simulink model "generic_IVS"  (R2024a)
settings: Solver=FixedStepDiscrete  StartTime=0.0  StopTime=inf  FixedStep=0.001  RelTol=1e-3  EnableMultiTasking=on
libraries: simulink x1, CarMaker4SL x1
(part 2 of 2)

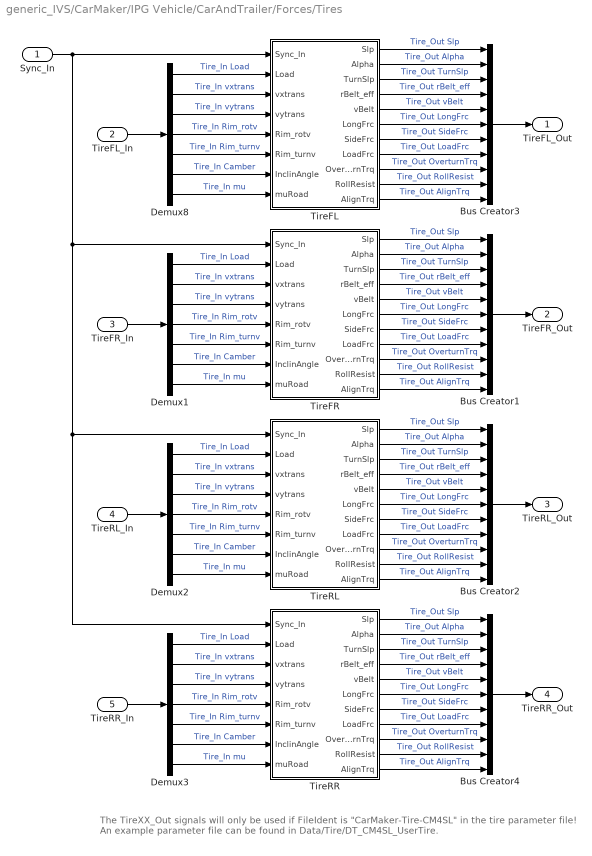
== system generic_IVS/CarMaker/IPG Vehicle/CarAndTrailer/Forces/Tires ==
  note: The TireXX_Out signals will only be used if FileIdent is "CarMaker-Tire-CM4SL" in the tire parameter file!
      | An example parameter file can be found in Data/Tire/DT_CM4SL_UserTire.
  Sync_In : Inport
  TireFL_In : Inport  Port=2
  TireFR_In : Inport  Port=3
  TireRL_In : Inport  Port=4
  TireRR_In : Inport  Port=5
  Bus Creator{1..4} (4 alike) : BusCreator  Inputs=11
  Demux{1..3,8} (4 alike) : Demux  Outputs=7
      settings: DisplayOption=none
  TireFL : Subsystem
  TireFR : Subsystem
  TireRL : Subsystem
  TireRR : Subsystem
  TireFL_Out : Outport  VectorParamsAs1DForOutWhenUnconnected=off
  TireFR_Out : Outport  Port=2  VectorParamsAs1DForOutWhenUnconnected=off
  TireRL_Out : Outport  Port=3  VectorParamsAs1DForOutWhenUnconnected=off
  TireRR_Out : Outport  Port=4  VectorParamsAs1DForOutWhenUnconnected=off
  wires:
  Sync_In/1 -> TireRR/1(Sync_In), TireRL/1(Sync_In), TireFR/1(Sync_In), TireFL/1(Sync_In)
  Bus Creator4/1 -> TireRR_Out/1
  Bus Creator2/1 -> TireRL_Out/1
  Bus Creator1/1 -> TireFR_Out/1
  Demux3/5 -> TireRR/6(Rim_turnv)  "Tire_In Rim_turnv"
  Demux3/4 -> TireRR/5(Rim_rotv)  "Tire_In Rim_rotv"
  Demux3/1 -> TireRR/2(Load)  "Tire_In Load"
  Demux3/7 -> TireRR/8(muRoad)  "Tire_In mu"
  Demux3/6 -> TireRR/7(InclinAngle)  "Tire_In Camber"
  Demux3/2 -> TireRR/3(vxtrans)  "Tire_In vxtrans"
  Demux3/3 -> TireRR/4(vytrans)  "Tire_In vytrans"
  TireRR/11(AlignTrq) -> Bus Creator4/11  "Tire_Out AlignTrq"
  TireRR/10(RollResist) -> Bus Creator4/10  "Tire_Out RollResist"
  TireRR/9(OverturnTrq) -> Bus Creator4/9  "Tire_Out OverturnTrq"
  TireRR/8(LoadFrc) -> Bus Creator4/8  "Tire_Out LoadFrc"
  TireRR/7(SideFrc) -> Bus Creator4/7  "Tire_Out SideFrc"
  TireRR/6(LongFrc) -> Bus Creator4/6  "Tire_Out LongFrc"
  TireRR/5(vBelt) -> Bus Creator4/5  "Tire_Out vBelt"
  TireRR/4(rBelt_eff) -> Bus Creator4/4  "Tire_Out rBelt_eff"
  TireRR/3(TurnSlp) -> Bus Creator4/3  "Tire_Out TurnSlp"
  TireRR/1(Slp) -> Bus Creator4/1  "Tire_Out Slp"
  TireRR/2(Alpha) -> Bus Creator4/2  "Tire_Out Alpha"
  Demux2/5 -> TireRL/6(Rim_turnv)  "Tire_In Rim_turnv"
  Demux2/4 -> TireRL/5(Rim_rotv)  "Tire_In Rim_rotv"
  Demux2/1 -> TireRL/2(Load)  "Tire_In Load"
  Demux2/7 -> TireRL/8(muRoad)  "Tire_In mu"
  Demux2/6 -> TireRL/7(InclinAngle)  "Tire_In Camber"
  Demux2/2 -> TireRL/3(vxtrans)  "Tire_In vxtrans"
  Demux2/3 -> TireRL/4(vytrans)  "Tire_In vytrans"
  TireRL/11(AlignTrq) -> Bus Creator2/11  "Tire_Out AlignTrq"
  TireRL/10(RollResist) -> Bus Creator2/10  "Tire_Out RollResist"
  TireRL/9(OverturnTrq) -> Bus Creator2/9  "Tire_Out OverturnTrq"
  TireRL/8(LoadFrc) -> Bus Creator2/8  "Tire_Out LoadFrc"
  TireRL/7(SideFrc) -> Bus Creator2/7  "Tire_Out SideFrc"
  TireRL/6(LongFrc) -> Bus Creator2/6  "Tire_Out LongFrc"
  TireRL/5(vBelt) -> Bus Creator2/5  "Tire_Out vBelt"
  TireRL/4(rBelt_eff) -> Bus Creator2/4  "Tire_Out rBelt_eff"
  TireRL/3(TurnSlp) -> Bus Creator2/3  "Tire_Out TurnSlp"
  TireRL/1(Slp) -> Bus Creator2/1  "Tire_Out Slp"
  TireRL/2(Alpha) -> Bus Creator2/2  "Tire_Out Alpha"
  Demux1/5 -> TireFR/6(Rim_turnv)  "Tire_In Rim_turnv"
  Demux1/4 -> TireFR/5(Rim_rotv)  "Tire_In Rim_rotv"
  Demux1/1 -> TireFR/2(Load)  "Tire_In Load"
  Demux1/7 -> TireFR/8(muRoad)  "Tire_In mu"
  Demux1/6 -> TireFR/7(InclinAngle)  "Tire_In Camber"
  Demux1/2 -> TireFR/3(vxtrans)  "Tire_In vxtrans"
  Demux1/3 -> TireFR/4(vytrans)  "Tire_In vytrans"
  TireFR/11(AlignTrq) -> Bus Creator1/11  "Tire_Out AlignTrq"
  TireFR/10(RollResist) -> Bus Creator1/10  "Tire_Out RollResist"
  TireFR/9(OverturnTrq) -> Bus Creator1/9  "Tire_Out OverturnTrq"
  TireFR/8(LoadFrc) -> Bus Creator1/8  "Tire_Out LoadFrc"
  TireFR/7(SideFrc) -> Bus Creator1/7  "Tire_Out SideFrc"
  TireFR/6(LongFrc) -> Bus Creator1/6  "Tire_Out LongFrc"
  TireFR/5(vBelt) -> Bus Creator1/5  "Tire_Out vBelt"
  TireFR/4(rBelt_eff) -> Bus Creator1/4  "Tire_Out rBelt_eff"
  TireFR/3(TurnSlp) -> Bus Creator1/3  "Tire_Out TurnSlp"
  TireFR/1(Slp) -> Bus Creator1/1  "Tire_Out Slp"
  TireFR/2(Alpha) -> Bus Creator1/2  "Tire_Out Alpha"
  Demux8/5 -> TireFL/6(Rim_turnv)  "Tire_In Rim_turnv"
  Demux8/4 -> TireFL/5(Rim_rotv)  "Tire_In Rim_rotv"
  TireFL_In/1 -> Demux8/1
  Demux8/1 -> TireFL/2(Load)  "Tire_In Load"
  Demux8/7 -> TireFL/8(muRoad)  "Tire_In mu"
  Demux8/6 -> TireFL/7(InclinAngle)  "Tire_In Camber"
  Demux8/2 -> TireFL/3(vxtrans)  "Tire_In vxtrans"
  Demux8/3 -> TireFL/4(vytrans)  "Tire_In vytrans"
  TireFL/11(AlignTrq) -> Bus Creator3/11  "Tire_Out AlignTrq"
  TireFL/10(RollResist) -> Bus Creator3/10  "Tire_Out RollResist"
  TireFL/9(OverturnTrq) -> Bus Creator3/9  "Tire_Out OverturnTrq"
  TireFL/8(LoadFrc) -> Bus Creator3/8  "Tire_Out LoadFrc"
  TireFL/7(SideFrc) -> Bus Creator3/7  "Tire_Out SideFrc"
  TireFL/6(LongFrc) -> Bus Creator3/6  "Tire_Out LongFrc"
  TireFL/5(vBelt) -> Bus Creator3/5  "Tire_Out vBelt"
  TireFL/4(rBelt_eff) -> Bus Creator3/4  "Tire_Out rBelt_eff"
  TireFL/3(TurnSlp) -> Bus Creator3/3  "Tire_Out TurnSlp"
  TireFL/1(Slp) -> Bus Creator3/1  "Tire_Out Slp"
  TireFL/2(Alpha) -> Bus Creator3/2  "Tire_Out Alpha"
  Bus Creator3/1 -> TireFL_Out/1
  TireFR_In/1 -> Demux1/1
  TireRL_In/1 -> Demux2/1
  TireRR_In/1 -> Demux3/1

== system generic_IVS/CarMaker/IPG Vehicle/CarAndTrailer/Forces/Vehicle Forces ==
  Sync_In : Inport
  Bus Creator1 : BusCreator  Inputs=12
  Bus Creator8 : BusCreator  Inputs=16
  BusCreator1 : BusCreator  Inputs=4
  BusCreator2 : BusCreator  Inputs=9
  Demux : Demux  Outputs=16
      settings: DisplayOption=none
  Demux1 : Demux  Outputs=12
      settings: DisplayOption=none
  Demux2 : Demux  Outputs=13
      settings: DisplayOption=none
  Forces : S-Function  FunctionName=CM_Sfun  Parameters='Forces'  SFunctionDeploymentMode=off  EnableBusSupport=off
  Terminator : Terminator
  Sync_Out : Outport  VectorParamsAs1DForOutWhenUnconnected=off
  Car.Virtual : Outport  Port=2  VectorParamsAs1DForOutWhenUnconnected=off
  Car.Aero : Outport  Port=3  VectorParamsAs1DForOutWhenUnconnected=off
  Car.Load : Outport  Port=4  VectorParamsAs1DForOutWhenUnconnected=off
  wires:
  BusCreator1/1 -> Terminator/1  "Aero IF (in)"
  Demux2/13 -> BusCreator2/9  "car Aero Trq_1 z"
  Demux2/12 -> BusCreator2/8  "car Aero Trq_1 y"
  Demux2/11 -> BusCreator2/7  "car Aero Trq_1 x"
  Demux2/10 -> BusCreator2/6  "car Aero Frc_1 z"
  Demux2/9 -> BusCreator2/5  "car Aero Frc_1 y"
  Demux2/8 -> BusCreator2/4  "car Aero Frc_1 x"
  Demux2/7 -> BusCreator2/3  "car Aero PoA_1 z"
  Demux2/6 -> BusCreator2/2  "car Aero PoA_1 y"
  Demux2/5 -> BusCreator2/1  "car Aero PoA_1 x"
  Demux2/4 -> BusCreator1/4  "car Aero tau_1"
  Demux2/3 -> BusCreator1/3  "car Aero ApproachVel_1 z"
  Demux2/2 -> BusCreator1/2  "car Aero ApproachVel_1 y"
  Demux2/1 -> BusCreator1/1  "car Aero ApproachVel_1 x"
  Demux/16 -> Bus Creator8/16  "Car Load_3 tz"
  Demux/15 -> Bus Creator8/15  "Car Load_3 ty"
  Demux/14 -> Bus Creator8/14  "Car Load_3 tx"
  Demux/13 -> Bus Creator8/13  "Car Load_3 mass"
  Demux1/12 -> Bus Creator1/12  "Car Virtual Trq_0 z"
  Demux1/11 -> Bus Creator1/11  "Car Virtual Trq_0 y"
  Demux1/10 -> Bus Creator1/10  "Car Virtual Trq_0 x"
  Demux1/9 -> Bus Creator1/9  "Car Virtual Trq_1 z"
  Demux1/8 -> Bus Creator1/8  "Car Virtual Trq_1 y"
  Demux1/7 -> Bus Creator1/7  "Car Virtual Trq_1 x"
  Demux1/6 -> Bus Creator1/6  "Car Virtual Frc_0 z"
  Demux1/5 -> Bus Creator1/5  "Car Virtual Frc_0 y"
  Demux1/4 -> Bus Creator1/4  "Car Virtual Frc_0 x"
  Sync_In/1 -> Forces/1
  Forces/1 -> Sync_Out/1
  BusCreator2/1 -> Car.Aero/1
  Demux1/1 -> Bus Creator1/1  "Car Virtual Frc_1 x"
  Demux1/2 -> Bus Creator1/2  "Car Virtual Frc_1 y"
  Demux1/3 -> Bus Creator1/3  "Car Virtual Frc_1 z"
  Forces/3 -> Demux2/1
  Forces/2 -> Demux1/1
  Bus Creator1/1 -> Car.Virtual/1
  Bus Creator8/1 -> Car.Load/1
  Demux/1 -> Bus Creator8/1  "Car Load_0 mass"
  Demux/2 -> Bus Creator8/2  "Car Load_0 tx"
  Demux/3 -> Bus Creator8/3  "Car Load_0 ty"
  Demux/4 -> Bus Creator8/4  "Car Load_0 tz"
  Demux/5 -> Bus Creator8/5  "Car Load_1 mass"
  Demux/6 -> Bus Creator8/6  "Car Load_1 tx"
  Demux/7 -> Bus Creator8/7  "Car Load_1 ty"
  Demux/8 -> Bus Creator8/8  "Car Load_1 tz"
  Demux/9 -> Bus Creator8/9  "Car Load_2 mass"
  Demux/10 -> Bus Creator8/10  "Car Load_2 tx"
  Demux/11 -> Bus Creator8/11  "Car Load_2 ty"
  Demux/12 -> Bus Creator8/12  "Car Load_2 tz"
  Forces/4 -> Demux/1

== system generic_IVS/CarMaker/IPG Vehicle/CarAndTrailer/Trailer/CreateBus Car.Hitch.FrcTrq ==
  In1 : Inport
  Bus Creator7 : BusCreator  Inputs=6
  Demux7 : Demux  Outputs=6
      settings: DisplayOption=none
  Out1 : Outport  VectorParamsAs1DForOutWhenUnconnected=off
  wires:
  In1/1 -> Demux7/1
  Bus Creator7/1 -> Out1/1
  Demux7/6 -> Bus Creator7/6  "Car Hitch Trq2Car z"
  Demux7/5 -> Bus Creator7/5  "Car Hitch Trq2Car y"
  Demux7/4 -> Bus Creator7/4  "Car Hitch Trq2Car x"
  Demux7/3 -> Bus Creator7/3  "Car Hitch Frc2Car z"
  Demux7/2 -> Bus Creator7/2  "Car Hitch Frc2Car y"
  Demux7/1 -> Bus Creator7/1  "Car Hitch Frc2Car x"

== system generic_IVS/CarMaker/IPG Vehicle/CarAndTrailer/Trailer/CreateBus Vhcl.Motion ==
  In1 : Inport
  BusCreator : BusCreator  Inputs=15
  Demux : Demux  Outputs=15
      settings: DisplayOption=none
  Out1 : Outport  VectorParamsAs1DForOutWhenUnconnected=off
  wires:
  Demux/15 -> BusCreator/15  "Vhcl YawAcc"
  Demux/14 -> BusCreator/14  "Vhcl YawVel"
  Demux/13 -> BusCreator/13  "Vhcl Yaw"
  Demux/12 -> BusCreator/12  "Vhcl PitchAcc"
  Demux/11 -> BusCreator/11  "Vhcl PitchVel"
  Demux/10 -> BusCreator/10  "Vhcl Pitch"
  Demux/9 -> BusCreator/9  "Vhcl RollAcc"
  Demux/8 -> BusCreator/8  "Vhcl RollVel"
  Demux/7 -> BusCreator/7  "Vhcl Roll"
  Demux/6 -> BusCreator/6  "Vhcl Hitch_Pos z"
  Demux/5 -> BusCreator/5  "Vhcl Hitch_Pos y"
  Demux/4 -> BusCreator/4  "Vhcl Hitch_Pos x"
  Demux/3 -> BusCreator/3  "Vhcl sRoad"
  Demux/2 -> BusCreator/2  "Vhcl Distance"
  Demux/1 -> BusCreator/1  "Vhcl v"
  In1/1 -> Demux/1
  BusCreator/1 -> Out1/1

== system generic_IVS/CarMaker/IPG Vehicle/CarAndTrailer/Trailer/CreateBus Vhcl.PoI ==
  In1 : Inport
  Bus Creator3 : BusCreator  Inputs=18
  Demux3 : Demux  Outputs=18
      settings: DisplayOption=none
  Out1 : Outport  VectorParamsAs1DForOutWhenUnconnected=off
  wires:
  Demux3/18 -> Bus Creator3/18  "Vhcl PoI_GCS Elev"
  Demux3/17 -> Bus Creator3/17  "Vhcl PoI_GCS Lat"
  Demux3/16 -> Bus Creator3/16  "Vhcl PoI_GCS Long"
  Demux3/15 -> Bus Creator3/15  "Vhcl PoI_Acc_1 z"
  Demux3/14 -> Bus Creator3/14  "Vhcl PoI_Acc_1 y"
  Demux3/13 -> Bus Creator3/13  "Vhcl PoI_Acc_1 x"
  Demux3/12 -> Bus Creator3/12  "Vhcl PoI_Vel_1 z"
  Demux3/11 -> Bus Creator3/11  "Vhcl PoI_Vel_1 y"
  Demux3/10 -> Bus Creator3/10  "Vhcl PoI_Vel_1 x"
  Demux3/9 -> Bus Creator3/9  "Vhcl PoI_Acc z"
  Demux3/8 -> Bus Creator3/8  "Vhcl PoI_Acc y"
  Demux3/7 -> Bus Creator3/7  "Vhcl PoI_Acc x"
  Demux3/6 -> Bus Creator3/6  "Vhcl PoI_Vel z"
  Demux3/5 -> Bus Creator3/5  "Vhcl PoI_Vel y"
  Demux3/4 -> Bus Creator3/4  "Vhcl PoI_Vel x"
  Demux3/3 -> Bus Creator3/3  "Vhcl PoI_Pos z"
  Demux3/2 -> Bus Creator3/2  "Vhcl PoI_Pos y"
  In1/1 -> Demux3/1
  Bus Creator3/1 -> Out1/1
  Demux3/1 -> Bus Creator3/1  "Vhcl PoI_Pos x"

== system generic_IVS/CarMaker/IPG Vehicle/CarAndTrailer/Trailer/CreateBus Vhcl.Steering ==
  In1 : Inport
  Bus Creator3 : BusCreator  Inputs=4
  Demux : Demux
      settings: DisplayOption=none
  Out1 : Outport  VectorParamsAs1DForOutWhenUnconnected=off
  wires:
  Bus Creator3/1 -> Out1/1
  Demux/1 -> Bus Creator3/1  "Vhcl Steering Ang"
  Demux/3 -> Bus Creator3/3  "Vhcl Steering AngAcc"
  Demux/2 -> Bus Creator3/2  "Vhcl Steering AngVel"
  Demux/4 -> Bus Creator3/4  "Vhcl Steering Trq"
  In1/1 -> Demux/1

== system generic_IVS/CarMaker/IPG Vehicle/CarAndTrailer/Trailer/CreateBus Vhcl.Wheel.FL ==
  In1 : Inport
  Bus Creator3 : BusCreator  Inputs=14
  Demux3 : Demux  Outputs=14
      settings: DisplayOption=none
  Out1 : Outport  VectorParamsAs1DForOutWhenUnconnected=off
  wires:
  Demux3/14 -> Bus Creator3/14  "Vhcl Wheel FL Trq_WhlBearing"
  Demux3/13 -> Bus Creator3/13  "Vhcl Wheel FL Trq_T2W"
  Demux3/12 -> Bus Creator3/12  "Vhcl Wheel FL SideSlip"
  Demux3/11 -> Bus Creator3/11  "Vhcl Wheel FL LongSlip"
  Demux3/10 -> Bus Creator3/10  "Vhcl Wheel FL vBelt"
  Demux3/9 -> Bus Creator3/9  "Vhcl Wheel FL Fz"
  Demux3/8 -> Bus Creator3/8  "Vhcl Wheel FL Fy"
  Demux3/7 -> Bus Creator3/7  "Vhcl Wheel FL Fx"
  Demux3/6 -> Bus Creator3/6  "Vhcl Wheel FL r_zxy z"
  Demux3/5 -> Bus Creator3/5  "Vhcl Wheel FL r_zxy y"
  Demux3/4 -> Bus Creator3/4  "Vhcl Wheel FL r_zxy x"
  Demux3/3 -> Bus Creator3/3  "Vhcl Wheel FL t z"
  Demux3/2 -> Bus Creator3/2  "Vhcl Wheel FL t y"
  In1/1 -> Demux3/1
  Bus Creator3/1 -> Out1/1
  Demux3/1 -> Bus Creator3/1  "Vhcl Wheel FL t x"

== system generic_IVS/CarMaker/IPG Vehicle/CarAndTrailer/Trailer/CreateBus Vhcl.Wheel.FR ==
  In1 : Inport
  Bus Creator3 : BusCreator  Inputs=14
  Demux3 : Demux  Outputs=14
      settings: DisplayOption=none
  Out1 : Outport  VectorParamsAs1DForOutWhenUnconnected=off
  wires:
  Demux3/14 -> Bus Creator3/14  "Vhcl Wheel FR Trq_WhlBearing"
  Demux3/13 -> Bus Creator3/13  "Vhcl Wheel FR Trq_T2W"
  Demux3/12 -> Bus Creator3/12  "Vhcl Wheel FR SideSlip"
  Demux3/11 -> Bus Creator3/11  "Vhcl Wheel FR LongSlip"
  Demux3/10 -> Bus Creator3/10  "Vhcl Wheel FR vBelt"
  Demux3/9 -> Bus Creator3/9  "Vhcl Wheel FR Fz"
  Demux3/8 -> Bus Creator3/8  "Vhcl Wheel FR Fy"
  Demux3/7 -> Bus Creator3/7  "Vhcl Wheel FR Fx"
  Demux3/6 -> Bus Creator3/6  "Vhcl Wheel FR r_zxy z"
  Demux3/5 -> Bus Creator3/5  "Vhcl Wheel FR r_zxy y"
  Demux3/4 -> Bus Creator3/4  "Vhcl Wheel FR r_zxy x"
  Demux3/3 -> Bus Creator3/3  "Vhcl Wheel FR t z"
  Demux3/2 -> Bus Creator3/2  "Vhcl Wheel FR t y"
  In1/1 -> Demux3/1
  Bus Creator3/1 -> Out1/1
  Demux3/1 -> Bus Creator3/1  "Vhcl Wheel FR t x"

== system generic_IVS/CarMaker/IPG Vehicle/CarAndTrailer/Trailer/CreateBus Vhcl.Wheel.RL ==
  In1 : Inport
  Bus Creator3 : BusCreator  Inputs=14
  Demux3 : Demux  Outputs=14
      settings: DisplayOption=none
  Out1 : Outport  VectorParamsAs1DForOutWhenUnconnected=off
  wires:
  Demux3/14 -> Bus Creator3/14  "Vhcl Wheel RL Trq_WhlBearing"
  Demux3/13 -> Bus Creator3/13  "Vhcl Wheel RL Trq_T2W"
  Demux3/12 -> Bus Creator3/12  "Vhcl Wheel RL SideSlip"
  Demux3/11 -> Bus Creator3/11  "Vhcl Wheel RL LongSlip"
  Demux3/10 -> Bus Creator3/10  "Vhcl Wheel RL vBelt"
  Demux3/9 -> Bus Creator3/9  "Vhcl Wheel RL Fz"
  Demux3/8 -> Bus Creator3/8  "Vhcl Wheel RL Fy"
  Demux3/7 -> Bus Creator3/7  "Vhcl Wheel RL Fx"
  Demux3/6 -> Bus Creator3/6  "Vhcl Wheel RL r_zxy z"
  Demux3/5 -> Bus Creator3/5  "Vhcl Wheel RL r_zxy y"
  Demux3/4 -> Bus Creator3/4  "Vhcl Wheel RL r_zxy x"
  Demux3/3 -> Bus Creator3/3  "Vhcl Wheel RL t z"
  Demux3/2 -> Bus Creator3/2  "Vhcl Wheel RL t y"
  In1/1 -> Demux3/1
  Bus Creator3/1 -> Out1/1
  Demux3/1 -> Bus Creator3/1  "Vhcl Wheel RL t x"

== system generic_IVS/CarMaker/IPG Vehicle/CarAndTrailer/Trailer/CreateBus Vhcl.Wheel.RR ==
  In1 : Inport
  Bus Creator3 : BusCreator  Inputs=14
  Demux3 : Demux  Outputs=14
      settings: DisplayOption=none
  Out1 : Outport  VectorParamsAs1DForOutWhenUnconnected=off
  wires:
  Demux3/14 -> Bus Creator3/14  "Vhcl Wheel RR Trq_WhlBearing"
  Demux3/13 -> Bus Creator3/13  "Vhcl Wheel RR Trq_T2W"
  Demux3/12 -> Bus Creator3/12  "Vhcl Wheel RR SideSlip"
  Demux3/11 -> Bus Creator3/11  "Vhcl Wheel RR LongSlip"
  Demux3/10 -> Bus Creator3/10  "Vhcl Wheel RR vBelt"
  Demux3/9 -> Bus Creator3/9  "Vhcl Wheel RR Fz"
  Demux3/8 -> Bus Creator3/8  "Vhcl Wheel RR Fy"
  Demux3/7 -> Bus Creator3/7  "Vhcl Wheel RR Fx"
  Demux3/6 -> Bus Creator3/6  "Vhcl Wheel RR r_zxy z"
  Demux3/5 -> Bus Creator3/5  "Vhcl Wheel RR r_zxy y"
  Demux3/4 -> Bus Creator3/4  "Vhcl Wheel RR r_zxy x"
  Demux3/3 -> Bus Creator3/3  "Vhcl Wheel RR t z"
  Demux3/2 -> Bus Creator3/2  "Vhcl Wheel RR t y"
  In1/1 -> Demux3/1
  Bus Creator3/1 -> Out1/1
  Demux3/1 -> Bus Creator3/1  "Vhcl Wheel RR t x"

== system generic_IVS/CarMaker/IPG Vehicle/CarAndTrailer/Forces/Suspension Forces/Suspension External Forces Update ==
  Bus Creator21 : BusCreator  Inputs=6
  Bus Creator22 : BusCreator  Inputs=4
  Bus Creator23 : BusCreator  Inputs=4
  From : From  TagVisibility=global
  Ground{32..39} (8 alike) : Ground
  Out1 : Outport
  wires:
  [D] -> Bus Creator21/4
  Ground36/1 -> Bus Creator22/1
  From/1 -> Bus Creator21/1
  [B] -> Bus Creator21/2
  Ground34/1 -> Bus Creator23/3
  Ground32/1 -> Bus Creator23/1
  [C] -> Bus Creator21/3
  Bus Creator23/1 -> Bus Creator21/5
  Ground33/1 -> Bus Creator23/2
  Bus Creator22/1 -> Bus Creator21/6
  Bus Creator21/1 -> Out1/1
  Ground35/1 -> Bus Creator23/4
  Ground39/1 -> Bus Creator22/4
  Ground38/1 -> Bus Creator22/3
  Ground37/1 -> Bus Creator22/2

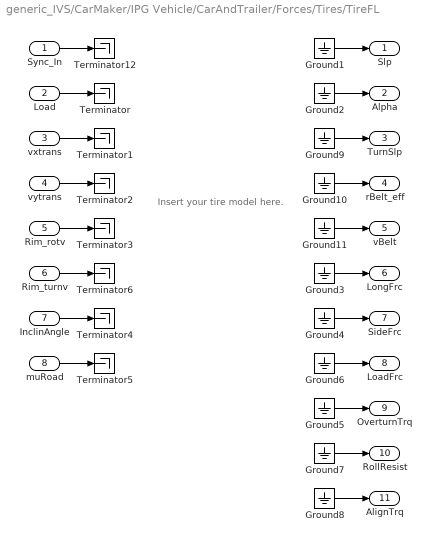
== system generic_IVS/CarMaker/IPG Vehicle/CarAndTrailer/Forces/Tires/TireFL ==
  note: Insert your tire model here.
  Sync_In : Inport
  Load : Inport  Port=2
  vxtrans : Inport  Port=3
  vytrans : Inport  Port=4
  Rim_rotv : Inport  Port=5
  Rim_turnv : Inport  Port=6
  InclinAngle : Inport  Port=7
  muRoad : Inport  Port=8
  Ground{1..11} (11 alike) : Ground
  Terminator{,1..6,12} (8 alike) : Terminator
  Slp : Outport  VectorParamsAs1DForOutWhenUnconnected=off
  Alpha : Outport  Port=2  VectorParamsAs1DForOutWhenUnconnected=off
  TurnSlp : Outport  Port=3  VectorParamsAs1DForOutWhenUnconnected=off
  rBelt_eff : Outport  Port=4  VectorParamsAs1DForOutWhenUnconnected=off
  vBelt : Outport  Port=5  VectorParamsAs1DForOutWhenUnconnected=off
  LongFrc : Outport  Port=6  VectorParamsAs1DForOutWhenUnconnected=off
  SideFrc : Outport  Port=7  VectorParamsAs1DForOutWhenUnconnected=off
  LoadFrc : Outport  Port=8  VectorParamsAs1DForOutWhenUnconnected=off
  OverturnTrq : Outport  Port=9  VectorParamsAs1DForOutWhenUnconnected=off
  RollResist : Outport  Port=10  VectorParamsAs1DForOutWhenUnconnected=off
  AlignTrq : Outport  Port=11  VectorParamsAs1DForOutWhenUnconnected=off
  wires:
  Ground11/1 -> vBelt/1
  Ground10/1 -> rBelt_eff/1
  Ground9/1 -> TurnSlp/1
  Rim_turnv/1 -> Terminator6/1
  Sync_In/1 -> Terminator12/1
  Ground2/1 -> Alpha/1
  Ground3/1 -> LongFrc/1
  Ground4/1 -> SideFrc/1
  Ground5/1 -> OverturnTrq/1
  vxtrans/1 -> Terminator1/1
  vytrans/1 -> Terminator2/1
  Rim_rotv/1 -> Terminator3/1
  InclinAngle/1 -> Terminator4/1
  muRoad/1 -> Terminator5/1
  Load/1 -> Terminator/1
  Ground1/1 -> Slp/1
  Ground6/1 -> LoadFrc/1
  Ground7/1 -> RollResist/1
  Ground8/1 -> AlignTrq/1

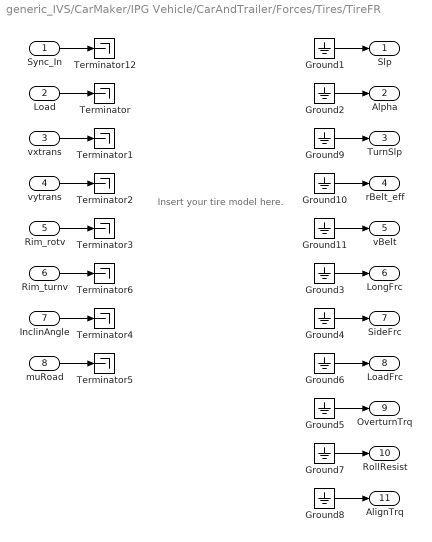
== system generic_IVS/CarMaker/IPG Vehicle/CarAndTrailer/Forces/Tires/TireFR ==
  note: Insert your tire model here.
  Sync_In : Inport
  Load : Inport  Port=2
  vxtrans : Inport  Port=3
  vytrans : Inport  Port=4
  Rim_rotv : Inport  Port=5
  Rim_turnv : Inport  Port=6
  InclinAngle : Inport  Port=7
  muRoad : Inport  Port=8
  Ground{1..11} (11 alike) : Ground
  Terminator{,1..6,12} (8 alike) : Terminator
  Slp : Outport  VectorParamsAs1DForOutWhenUnconnected=off
  Alpha : Outport  Port=2  VectorParamsAs1DForOutWhenUnconnected=off
  TurnSlp : Outport  Port=3  VectorParamsAs1DForOutWhenUnconnected=off
  rBelt_eff : Outport  Port=4  VectorParamsAs1DForOutWhenUnconnected=off
  vBelt : Outport  Port=5  VectorParamsAs1DForOutWhenUnconnected=off
  LongFrc : Outport  Port=6  VectorParamsAs1DForOutWhenUnconnected=off
  SideFrc : Outport  Port=7  VectorParamsAs1DForOutWhenUnconnected=off
  LoadFrc : Outport  Port=8  VectorParamsAs1DForOutWhenUnconnected=off
  OverturnTrq : Outport  Port=9  VectorParamsAs1DForOutWhenUnconnected=off
  RollResist : Outport  Port=10  VectorParamsAs1DForOutWhenUnconnected=off
  AlignTrq : Outport  Port=11  VectorParamsAs1DForOutWhenUnconnected=off
  wires:
  Ground11/1 -> vBelt/1
  Ground10/1 -> rBelt_eff/1
  Ground9/1 -> TurnSlp/1
  Rim_turnv/1 -> Terminator6/1
  Sync_In/1 -> Terminator12/1
  Ground2/1 -> Alpha/1
  Ground3/1 -> LongFrc/1
  Ground4/1 -> SideFrc/1
  Ground5/1 -> OverturnTrq/1
  vxtrans/1 -> Terminator1/1
  vytrans/1 -> Terminator2/1
  Rim_rotv/1 -> Terminator3/1
  InclinAngle/1 -> Terminator4/1
  muRoad/1 -> Terminator5/1
  Load/1 -> Terminator/1
  Ground1/1 -> Slp/1
  Ground6/1 -> LoadFrc/1
  Ground7/1 -> RollResist/1
  Ground8/1 -> AlignTrq/1

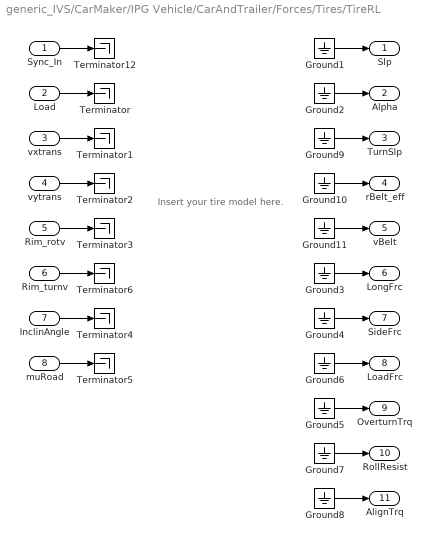
== system generic_IVS/CarMaker/IPG Vehicle/CarAndTrailer/Forces/Tires/TireRL ==
  note: Insert your tire model here.
  Sync_In : Inport
  Load : Inport  Port=2
  vxtrans : Inport  Port=3
  vytrans : Inport  Port=4
  Rim_rotv : Inport  Port=5
  Rim_turnv : Inport  Port=6
  InclinAngle : Inport  Port=7
  muRoad : Inport  Port=8
  Ground{1..11} (11 alike) : Ground
  Terminator{,1..6,12} (8 alike) : Terminator
  Slp : Outport  VectorParamsAs1DForOutWhenUnconnected=off
  Alpha : Outport  Port=2  VectorParamsAs1DForOutWhenUnconnected=off
  TurnSlp : Outport  Port=3  VectorParamsAs1DForOutWhenUnconnected=off
  rBelt_eff : Outport  Port=4  VectorParamsAs1DForOutWhenUnconnected=off
  vBelt : Outport  Port=5  VectorParamsAs1DForOutWhenUnconnected=off
  LongFrc : Outport  Port=6  VectorParamsAs1DForOutWhenUnconnected=off
  SideFrc : Outport  Port=7  VectorParamsAs1DForOutWhenUnconnected=off
  LoadFrc : Outport  Port=8  VectorParamsAs1DForOutWhenUnconnected=off
  OverturnTrq : Outport  Port=9  VectorParamsAs1DForOutWhenUnconnected=off
  RollResist : Outport  Port=10  VectorParamsAs1DForOutWhenUnconnected=off
  AlignTrq : Outport  Port=11  VectorParamsAs1DForOutWhenUnconnected=off
  wires:
  Ground11/1 -> vBelt/1
  Ground10/1 -> rBelt_eff/1
  Ground9/1 -> TurnSlp/1
  Rim_turnv/1 -> Terminator6/1
  Sync_In/1 -> Terminator12/1
  Ground2/1 -> Alpha/1
  Ground3/1 -> LongFrc/1
  Ground4/1 -> SideFrc/1
  Ground5/1 -> OverturnTrq/1
  vxtrans/1 -> Terminator1/1
  vytrans/1 -> Terminator2/1
  Rim_rotv/1 -> Terminator3/1
  InclinAngle/1 -> Terminator4/1
  muRoad/1 -> Terminator5/1
  Load/1 -> Terminator/1
  Ground1/1 -> Slp/1
  Ground6/1 -> LoadFrc/1
  Ground7/1 -> RollResist/1
  Ground8/1 -> AlignTrq/1

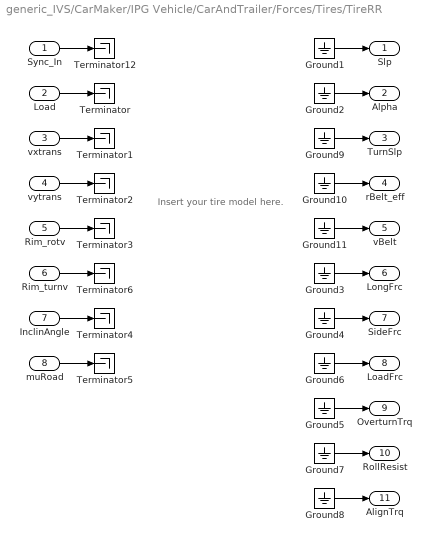
== system generic_IVS/CarMaker/IPG Vehicle/CarAndTrailer/Forces/Tires/TireRR ==
  note: Insert your tire model here.
  Sync_In : Inport
  Load : Inport  Port=2
  vxtrans : Inport  Port=3
  vytrans : Inport  Port=4
  Rim_rotv : Inport  Port=5
  Rim_turnv : Inport  Port=6
  InclinAngle : Inport  Port=7
  muRoad : Inport  Port=8
  Ground{1..11} (11 alike) : Ground
  Terminator{,1..6,12} (8 alike) : Terminator
  Slp : Outport  VectorParamsAs1DForOutWhenUnconnected=off
  Alpha : Outport  Port=2  VectorParamsAs1DForOutWhenUnconnected=off
  TurnSlp : Outport  Port=3  VectorParamsAs1DForOutWhenUnconnected=off
  rBelt_eff : Outport  Port=4  VectorParamsAs1DForOutWhenUnconnected=off
  vBelt : Outport  Port=5  VectorParamsAs1DForOutWhenUnconnected=off
  LongFrc : Outport  Port=6  VectorParamsAs1DForOutWhenUnconnected=off
  SideFrc : Outport  Port=7  VectorParamsAs1DForOutWhenUnconnected=off
  LoadFrc : Outport  Port=8  VectorParamsAs1DForOutWhenUnconnected=off
  OverturnTrq : Outport  Port=9  VectorParamsAs1DForOutWhenUnconnected=off
  RollResist : Outport  Port=10  VectorParamsAs1DForOutWhenUnconnected=off
  AlignTrq : Outport  Port=11  VectorParamsAs1DForOutWhenUnconnected=off
  wires:
  Ground11/1 -> vBelt/1
  Ground10/1 -> rBelt_eff/1
  Ground9/1 -> TurnSlp/1
  Rim_turnv/1 -> Terminator6/1
  Sync_In/1 -> Terminator12/1
  Ground2/1 -> Alpha/1
  Ground3/1 -> LongFrc/1
  Ground4/1 -> SideFrc/1
  Ground5/1 -> OverturnTrq/1
  vxtrans/1 -> Terminator1/1
  vytrans/1 -> Terminator2/1
  Rim_rotv/1 -> Terminator3/1
  InclinAngle/1 -> Terminator4/1
  muRoad/1 -> Terminator5/1
  Load/1 -> Terminator/1
  Ground1/1 -> Slp/1
  Ground6/1 -> LoadFrc/1
  Ground7/1 -> RollResist/1
  Ground8/1 -> AlignTrq/1

== stateflow chart generic_IVS/CarMaker/Subsystem/Day3/Chart ==
  (default) -> (junction 1)
  (junction 1) -> (junction 3) [order 1] : [i<99]
      | {i = i + 1;}
  (junction 1) -> (junction 7) [order 2] : {i=0;}
  (junction 3) -> (junction 5)
  (junction 5) -> (junction 7)
  (junction 7) -> (junction 10)
  (junction 10) -> (junction 12) [order 1] : [rem(i,50) == 0]
      | {do_Logic;}
  (junction 10) -> (junction 18) [order 2]
  (junction 12) -> (junction 16)
  (junction 16) -> (junction 18)
  (junction 18) -> (junction 21)
  data: i local =0
  events: do_Logic output FUNCTION_CALL_EVENT
